simulink model "GuidanceLaw"  (R2023b)
settings: Solver=ode4  StartTime=0.0  StopTime=400  FixedStep=0.05  RelTol=1e-3
values from neighbouring files (symbols this model uses):
  APCMD_TYPE : value not decoded    [apDataDictionary.sldd]
  missionRoutePlan_struct = struct(      'validWpNum_u8', uint8(5),      'missionRoute_struct', repmat(wpDefault_struct, double(maxWpNum_u8), 1))    [initMissionRoutePlan_MC.m]
  MSSN_TYPE : value not decoded    [apDataDictionary.sldd]
  setPoint_struct = struct('lat_deg_d',double(31.200000),'lon_deg_d',double(121.500000),'alt_m_f',single(100),'yaw_deg_f',single(0))    [APTest.m]
undefined symbols (not defined in the file or in its folder): apParams
libraries: simulink x13, simulink_extras x3
(part 5 of 7)

== matlab function GuidanceLaw/Subsystem/wpMssnHandle/CrsTransform/geoToLocalNEU ==
  data: curGeo_struct input; curPosNEU_m_f output; preWpGeo_struct input; curWpGeo_struct input; nextWpGeo_struct input; segSwitch_b input; preWpNEU_m_f output; curWpNEU_m_f output; nextWpNEU_m_f output; newOriOldNEU_m_f output
function [curPosNEU_m_f, preWpNEU_m_f, curWpNEU_m_f, nextWpNEU_m_f, newOriOldNEU_m_f] = geoToLocalNEU(curGeo_struct, preWpGeo_struct, curWpGeo_struct, ...
    nextWpGeo_struct, segSwitch_b)
%#codegen
%
% 功能：
% 1. 以当前执行航点作为局部NEU坐标系原点；
% 2. 将当前位置、上一航点、当前航点和下一航点转换到局部NEU；
% 3. 航段切换时计算新原点在旧局部坐标系中的位置。
%
% 输入经纬高结构体字段：
% lat_deg_d：纬度，deg，double；
% lon_deg_d：经度，deg，double；
% alt_m_f：高度，m，single。

%% 保存上一周期实际使用的局部坐标原点

persistent lastOriginLat_deg_d
persistent lastOriginLon_deg_d
persistent lastOriginAlt_m_f
persistent originInitialized_b

if isempty(originInitialized_b)
    lastOriginLat_deg_d = double(0.0);
    lastOriginLon_deg_d = double(0.0);
    lastOriginAlt_m_f = single(0.0);
    originInitialized_b = false;
end


%% 当前局部坐标系原点

originLL_deg_d = [curWpGeo_struct.lat_deg_d, curWpGeo_struct.lon_deg_d];

originAlt_m_f = curWpGeo_struct.alt_m_f;

if ~originInitialized_b
    % 第一次运行没有旧坐标系，此时不需要平移轨迹状态
    lastOriginLat_deg_d = originLL_deg_d(1);
    lastOriginLon_deg_d = originLL_deg_d(2);
    lastOriginAlt_m_f = originAlt_m_f;
    originInitialized_b = true;
end

%% 飞机当前位置

curLL_deg_d = [curGeo_struct.lat_deg_d, curGeo_struct.lon_deg_d];

curPosNE_m_f = getDistanceNE(originLL_deg_d, curLL_deg_d);

curPosNEU_m_f = single(zeros(3,1));
curPosNEU_m_f(1) = curPosNE_m_f(1);
curPosNEU_m_f(2) = curPosNE_m_f(2);
curPosNEU_m_f(3) = curGeo_struct.alt_m_f - originAlt_m_f;

%% 上一航点

preWpLL_deg_d = [preWpGeo_struct.lat_deg_d, preWpGeo_struct.lon_deg_d];

preWpNE_m_f = getDistanceNE(originLL_deg_d, preWpLL_deg_d);

preWpNEU_m_f = single(zeros(3,1));
preWpNEU_m_f(1) = preWpNE_m_f(1);
preWpNEU_m_f(2) = preWpNE_m_f(2);
preWpNEU_m_f(3) = preWpGeo_struct.alt_m_f - originAlt_m_f;

%% 当前执行航点

% 当前执行航点就是局部坐标系原点。
curWpNEU_m_f = single(zeros(3,1));

%% 下一航点

nextWpLL_deg_d = [nextWpGeo_struct.lat_deg_d, nextWpGeo_struct.lon_deg_d];

nextWpNE_m_f = getDistanceNE(originLL_deg_d, nextWpLL_deg_d);

nextWpNEU_m_f = single(zeros(3,1));
nextWpNEU_m_f(1) = nextWpNE_m_f(1);
nextWpNEU_m_f(2) = nextWpNE_m_f(2);
nextWpNEU_m_f(3) = nextWpGeo_struct.alt_m_f - originAlt_m_f;

%% 新原点在旧局部坐标系中的位置

newOriOldNEU_m_f = single(zeros(3,1));

if segSwitch_b
    oldOriginLL_deg_d = [lastOriginLat_deg_d, lastOriginLon_deg_d];

    newOriginOldNE_m_f = getDistanceNE(oldOriginLL_deg_d, originLL_deg_d);

    newOriOldNEU_m_f(1) = single(newOriginOldNE_m_f(1));
    newOriOldNEU_m_f(2) = single(newOriginOldNE_m_f(2));
    newOriOldNEU_m_f(3) = originAlt_m_f - lastOriginAlt_m_f;
end

%% 保存本周期实际原点，供下一次切换使用

lastOriginLat_deg_d = originLL_deg_d(1);
lastOriginLon_deg_d = originLL_deg_d(2);
lastOriginAlt_m_f = originAlt_m_f;

end

== matlab function GuidanceLaw/Subsystem/wpMssnHandle/WpUpdate/WaypointSelector ==
  data: route_struct input; preWp_struct output Bus: wayPointBus; validWpNum_u8 input; curWpIdx_u8 input; curWp_struct output Bus: wayPointBus; nextWp_struct output Bus: wayPointBus
function [preWp_struct, curWp_struct, nextWp_struct] = WaypointSelector(route_struct, validWpNum_u8, curWpIdx_u8)
%#codegen
preWp_struct  = route_struct(1);
curWp_struct  = route_struct(1);
nextWp_struct = route_struct(1);

% 要求初始执行航点序列为2
if validWpNum_u8 < uint8(2) || curWpIdx_u8 < uint8(2)
    preWp_struct.wpType_u8  = WP_TYPE.INVALID_WP;
    curWp_struct.wpType_u8  = WP_TYPE.INVALID_WP;
    nextWp_struct.wpType_u8 = WP_TYPE.INVALID_WP;
    return;
end

idx_d = min(curWpIdx_u8,validWpNum_u8);
preWp_struct = route_struct(idx_d - uint8(1));
curWp_struct = route_struct(idx_d);

if idx_d < validWpNum_u8
    nextWp_struct = route_struct(idx_d + uint8(1));
else 
    nextWp_struct = curWp_struct;
    nextWp_struct.wpType_u8 = WP_TYPE.INVALID_WP;
end
end

== matlab function GuidanceLaw/Subsystem/wpMssnHandle/WaypointArrivalState/hoverPosJudge/conditionHoldJudge ==
  data: condition_b input; hoverPosJudge_b output; reset_b input; dt_s_f input; holdTimeCond_s_f input
function hoverPosJudge_b = conditionHoldJudge(condition_b, reset_b, dt_s_f, holdTimeCond_s_f)
%#codegen
%
% 条件连续保持时间判定
%
% 输入：
% condition_b           当前周期原始综合条件；
% reset_b               航段切换复位信号；
% dt_s_f                函数运行周期，s；
% holdTimeCond_s_f      条件需要连续保持的时间，s。
%
% 输出：
% hoverPosJudge_b       条件连续保持时间满足标志。

persistent holdElapsedTimeState_s_f

%% 状态初始化
if isempty(holdElapsedTimeState_s_f)
    holdElapsedTimeState_s_f = single(0.0);
end

%% 输入保护
dtValid_s_f = max(single(dt_s_f), single(0.0));
holdTimeValid_s_f = max(single(holdTimeCond_s_f), single(0.0));

%% 复位内部历史状态
if reset_b
    holdElapsedTimeState_s_f = single(0.0);
end

%% 本周期条件更新
if ~condition_b
    % 条件不成立，连续保持过程立即中断
    holdElapsedTimeState_s_f = single(0.0);
    hoverPosJudge_b = false;

elseif holdTimeValid_s_f <= single(0.0)
    % 无保持时间要求，当前周期条件成立即满足
    holdElapsedTimeState_s_f = single(0.0);
    hoverPosJudge_b = true;

else
    % 当前周期条件成立，立即累计一个执行周期
    elapsedTimeNext_s_f = holdElapsedTimeState_s_f + dtValid_s_f;

    % 达到目标时间后饱和，避免持续累加
    if elapsedTimeNext_s_f >= holdTimeValid_s_f
        holdElapsedTimeState_s_f = holdTimeValid_s_f;
        hoverPosJudge_b = true;
    else
        holdElapsedTimeState_s_f = elapsedTimeNext_s_f;
        hoverPosJudge_b = false;
    end
end

end

== stateflow chart GuidanceLaw/Subsystem/wpMssnHandle/WaypointArrivalState/ArrivalJudgeSelect ==
  state ACTIVE
    entry:
    judgeMethod_u8 = uint8(0);
    hoverPosJudgeEn_b = false;
    hoverYawJudgeEn_b = false;
    mcLineJudgeEn_b = false;
    fwLineJudgeEn_b = false;
    cirJudgeEn_b = false;
    state HOVER_POSITION
      entry:
      judgeMethod_u8 = uint8(1);
      hoverPosJudgeEn_b = true;
    note: 偏航角类型
        | 0：航向对准
        | 1：航点指定
        | 2：指向航点
    state HOVER_YAW_ALIGN
      entry:
      judgeMethod_u8 = uint8(2);
      hoverYawJudgeEn_b = true;
    state MC_LINE
      entry:
      judgeMethod_u8 = uint8(3);
      mcLineJudgeEn_b = true;
    state FW_LINE
      entry:
      judgeMethod_u8 = uint8(4);
      fwLineJudgeEn_b = true;
    state FW_CIR
      entry:
      judgeMethod_u8 = uint8(5);
      cirJudgeEn_b = true;
    state INVALID
      entry:
      judgeMethod_u8 = uint8(0);
    (junction 34) -> HOVER_POSITION [order 1] : [(curWp_struct.wpType_u8 == WP_TYPE.MC_TAKEOFF_WP && mssnType_u8 == MSSN_TYPE.VERTICAL_TAKEOFF) ||...
        |  (curWp_struct.wpType_u8 == WP_TYPE.MC_LAND_WP && preWp_struct.wpType_u8 ~= WP_TYPE.MC_LAND_WP)]
    (junction 34) -> HOVER_YAW_ALIGN [order 2] : [(curWp_struct.wpType_u8 == WP_TYPE.MC_TAKEOFF_WP && mssnType_u8 == MSSN_TYPE.ROUTE_FLIGHT) ||...
        | (curWp_struct.wpType_u8 == WP_TYPE.MC_LINE_WP && curWp_struct.fastWp_b == false)]
    (default) -> (junction 34)
    (junction 34) -> MC_LINE [order 3] : [curWp_struct.wpType_u8 == WP_TYPE.MC_LINE_WP && curWp_struct.fastWp_b == true]
    (junction 34) -> FW_LINE [order 4] : [curWp_struct.wpType_u8 == WP_TYPE.FW_LINE_WP &&...
        | mssnType_u8 ~=MSSN_TYPE.AUTO_FORWARD_TILT]
    (junction 34) -> FW_CIR [order 5] : [curWp_struct.wpType_u8 == WP_TYPE.FW_CIR_WP]
    (junction 34) -> INVALID [order 6]
  (default) -> ACTIVE
  ACTIVE -> ACTIVE : [segSwitch_b]
  data: curWp_struct input Bus: localNEUWpBus size=1; mssnType_u8 input size=1; segSwitch_b input boolean size=1; judgeMethod_u8 output uint8 size=1; hoverPosJudgeEn_b output boolean size=1; hoverYawJudgeEn_b output boolean size=1; mcLineJudgeEn_b output boolean size=1; fwLineJudgeEn_b output boolean size=1; cirJudgeEn_b output boolean size=1; nextWp_struct input Bus: localNEUWpBus size=1; preWp_struct input Bus: localNEUWpBus size=1

== matlab function GuidanceLaw/Subsystem/wpMssnHandle/WaypointArrivalState/hoverYawJudge/conditionHoldJudge ==
  data: condition_b input; hoverPosJudge_b output; reset_b input; dt_s_f input; holdTimeCond_s_f input
function hoverPosJudge_b = conditionHoldJudge(condition_b, reset_b, dt_s_f, holdTimeCond_s_f)
%#codegen
%
% 条件连续保持时间判定
%
% 输入：
% condition_b           当前周期原始综合条件；
% reset_b               航段切换复位信号；
% dt_s_f                函数运行周期，s；
% holdTimeCond_s_f      条件需要连续保持的时间，s。
%
% 输出：
% hoverPosJudge_b       条件连续保持时间满足标志。

persistent holdElapsedTimeState_s_f

%% 状态初始化
if isempty(holdElapsedTimeState_s_f)
    holdElapsedTimeState_s_f = single(0.0);
end

%% 输入保护
dtValid_s_f = max(single(dt_s_f), single(0.0));
holdTimeValid_s_f = max(single(holdTimeCond_s_f), single(0.0));

%% 复位内部历史状态
if reset_b
    holdElapsedTimeState_s_f = single(0.0);
end

%% 本周期条件更新
if ~condition_b
    % 条件不成立，连续保持过程立即中断
    holdElapsedTimeState_s_f = single(0.0);
    hoverPosJudge_b = false;

elseif holdTimeValid_s_f <= single(0.0)
    % 无保持时间要求，当前周期条件成立即满足
    holdElapsedTimeState_s_f = single(0.0);
    hoverPosJudge_b = true;

else
    % 当前周期条件成立，立即累计一个执行周期
    elapsedTimeNext_s_f = holdElapsedTimeState_s_f + dtValid_s_f;

    % 达到目标时间后饱和，避免持续累加
    if elapsedTimeNext_s_f >= holdTimeValid_s_f
        holdElapsedTimeState_s_f = holdTimeValid_s_f;
        hoverPosJudge_b = true;
    else
        holdElapsedTimeState_s_f = elapsedTimeNext_s_f;
        hoverPosJudge_b = false;
    end
end

end

== stateflow chart GuidanceLaw/Subsystem/wpMssnHandle/WaypointArrivalState/hoverYawJudge/HoverPosReachStateflow ==
  state WAIT_POSITION
    entry:
    isHoverPosReach_b = false;
  state POS_REACHED
    entry:
    isHoverPosReach_b = true;
  (default) -> (junction 13)
  (junction 13) -> POS_REACHED [order 1] : [hoverPosJudge_b]
  (junction 13) -> WAIT_POSITION [order 2]
  POS_REACHED -> (junction 13) : [reset_b]
  WAIT_POSITION -> POS_REACHED : [hoverPosJudge_b]
  data: hoverPosJudge_b input boolean size=1; reset_b input boolean size=1; isHoverPosReach_b output boolean size=1

== matlab function GuidanceLaw/Subsystem/wpMssnHandle/WaypointArrivalState/hoverYawJudge/YawAlignJudge/YawJudgeAlgorithmBlock ==
  data: curPosNE_m_f input; nextWpNE_m_f input; hoverYawJudge_b output boolean; curYaw_deg_f input; nextWpYawType_u8 input; nextWpYaw_deg_f input; reset_b input; dt_s_f input; yawErrAccept_deg_f input; holdTimeYaw_s_f input; minYawDirDist_m_f input; yawCmd_deg_f output; curWpNE_m_f input
function [hoverYawJudge_b, yawCmd_deg_f] = hoverYawAlignJudge(curPosNE_m_f, nextWpNE_m_f, curYaw_deg_f, nextWpYawType_u8, nextWpYaw_deg_f, reset_b, dt_s_f, ...
    yawErrAccept_deg_f, holdTimeYaw_s_f, minYawDirDist_m_f, curWpNE_m_f)
%#codegen
%
% 悬停位置到达后的目标航向生成与航向对准判定
%
% 下一航点偏航角类型：
% 0：航向对准——当前航点指向下一航点；
% 1：指向航点——位置到达时飞机位置指向下一航点；
% 2：航点指定——下一航点设定的偏航角。

persistent yawCmdState_deg_f
persistent yawCmdLockedState_b
persistent yawHoldTimeState_s_f
persistent yawReachedState_b

%% 状态初始化
if isempty(yawCmdState_deg_f)
    yawCmdState_deg_f = single(0.0);
    yawCmdLockedState_b = false;
    yawHoldTimeState_s_f = single(0.0);
    yawReachedState_b = false;
end

%% 参数保护
dtValid_s_f = max(dt_s_f, single(0.0));

yawErrAcceptValid_deg_f = min(max(yawErrAccept_deg_f, single(0.0)), single(180.0));

holdTimeYawValid_s_f = max(holdTimeYaw_s_f, single(0.0));

minYawDirDistValid_m_f = max(minYawDirDist_m_f, single(0.0));

%% 航段切换复位
% 只清除旧状态，随后仍处理当前拍。
if reset_b
    yawCmdState_deg_f = cldWrap180(curYaw_deg_f);
    yawCmdLockedState_b = false;
    yawHoldTimeState_s_f = single(0.0);
    yawReachedState_b = false;
end

%% 目标航向计算与锁存
if ~yawCmdLockedState_b

    % 位置首次到达，仅在当前拍计算一次目标航向。
    switch uint8(nextWpYawType_u8)

        case uint8(0)
            %% 航向对准
            % 当前航点为局部坐标系原点。
            yawDirN_m_f = nextWpNE_m_f(1) - curWpNE_m_f(1);
            yawDirE_m_f = nextWpNE_m_f(2) - curWpNE_m_f(2);

            yawCmdState_deg_f = directionNEToYaw(yawDirN_m_f, yawDirE_m_f, curYaw_deg_f, minYawDirDistValid_m_f);

        case uint8(1)
            %% 航点指定
            yawCmdState_deg_f = cldWrap180(nextWpYaw_deg_f);

        case uint8(2)

            %% 指向航点
            % 使用位置到达当前拍的飞机位置计算一次。
            yawDirN_m_f = nextWpNE_m_f(1) - curPosNE_m_f(1);

            yawDirE_m_f = nextWpNE_m_f(2) - curPosNE_m_f(2);

            yawCmdState_deg_f = directionNEToYaw(yawDirN_m_f, yawDirE_m_f, curYaw_deg_f, minYawDirDistValid_m_f);
            
        otherwise
            %% 无效偏航类型
            yawCmdState_deg_f = cldWrap180(curYaw_deg_f);
    end

    % 目标航向计算完成后立即锁存。
    yawCmdLockedState_b = true;
end

%% 输出锁存后的目标航向
yawCmd_deg_f = yawCmdState_deg_f;

%% 航向误差计算
yawErr_deg_f = cldWrap180(yawCmdState_deg_f - curYaw_deg_f);

yawCondition_b = yawCmdLockedState_b && abs(yawErr_deg_f) <= yawErrAcceptValid_deg_f;

%% 航向连续保持判定
if ~yawReachedState_b

    if ~yawCondition_b
        yawHoldTimeState_s_f = single(0.0);

    elseif holdTimeYawValid_s_f <= single(0.0)
        yawReachedState_b = true;

    else
        % 当前拍满足条件，立即累计一个dt。
        yawHoldTimeState_s_f = min(yawHoldTimeState_s_f + dtValid_s_f, holdTimeYawValid_s_f);

        yawReachedState_b = yawHoldTimeState_s_f >= holdTimeYawValid_s_f;
    end
end

%% 输出航向对准锁存结果
hoverYawJudge_b = yawReachedState_b;

end


function yaw_deg_f = directionNEToYaw(directionN_m_f, directionE_m_f, fallbackYaw_deg_f, minDirectionDist_m_f)
%#codegen
%
% NE方向向量转换为航向角：
% 北向0 deg，东向90 deg。

directionDistSq_m2_f = directionN_m_f * directionN_m_f + directionE_m_f * directionE_m_f;

minDirectionDistSq_m2_f = minDirectionDist_m_f * minDirectionDist_m_f;

if directionDistSq_m2_f > minDirectionDistSq_m2_f
    radToDeg_f = single(180.0 / pi);

    yaw_deg_f = atan2(directionE_m_f, directionN_m_f) * radToDeg_f;

    yaw_deg_f = cldWrap180(yaw_deg_f);
else
    % 水平向量过小，保持位置到达时的当前航向。
    yaw_deg_f = cldWrap180(single(fallbackYaw_deg_f));
end

end

== matlab function GuidanceLaw/Subsystem/wpMssnHandle/WaypointArrivalState/mcLineJudge/JudgeAlgorithm ==
  data: curPosNE_m_f input; mcLineJudge_b output; preWpNE_m_f input; curWpNE_m_f input; nextWpNE_m_f input; maxRouteSpeed_mps_f input; maxLatAcc_mps2_f input; minJudgeDist_m_f input; maxJudgeDist_m_f input; segmentLimitRatio_f input; reset_b input
function mcLineJudge_b = mcLineJudge(curPosNE_m_f, preWpNE_m_f, curWpNE_m_f, nextWpNE_m_f, maxRouteSpeed_mps_f, maxLatAcc_mps2_f, minJudgeDist_m_f, maxJudgeDist_m_f, segmentLimitRatio_f, reset_b)
%#codegen
%
% 旋翼直线航点提前分界面判定。
%
% 与轨迹生成器共用computeMcTurnConstraint：
% 1. maxRouteSpeed_mps_f只作为最大速度，不再作为固定转弯速度；
% 2. 根据A-B-C转角、横向加速度和可用提前距离计算动态航点通过速度；
% 3. 本模块仅使用其中的judgeDist_m_f确定分界面；
% 4. 轨迹生成器使用同一judgeDist和passSpeed提前减速，二者保持一致。
%
% geometryState_f：
% 1 提前判定距离，m
% 2 A->B单位方向北向分量
% 3 A->B单位方向东向分量
% 4 B点在A->B单位方向上的投影，m

persistent completeState_b
persistent geometryState_f
persistent initialized_b

smallValue_m_f = single(0.001);

if isempty(initialized_b)
    completeState_b = false;
    geometryState_f = single(zeros(4,1));
    initialized_b = false;
end

%% 新航段几何计算并冻结
if reset_b || ~initialized_b
    completeState_b = false;
    geometryState_f = single(zeros(4,1));

    inVecNE_m_f = curWpNE_m_f - preWpNE_m_f;
    inLength_m_f = norm(inVecNE_m_f);
    shortLineThreshold_m_f = max(max(minJudgeDist_m_f, single(0.0)), smallValue_m_f);

    if inLength_m_f <= shortLineThreshold_m_f
        % 当前航段太短，直接判定完成。
        completeState_b = true;
    else
        inDirNE_f = inVecNE_m_f / inLength_m_f;

        [judgeDist_m_f, ~] = computeMcTurnConstraint(preWpNE_m_f, curWpNE_m_f, nextWpNE_m_f, maxRouteSpeed_mps_f, maxLatAcc_mps2_f, ...
            minJudgeDist_m_f, maxJudgeDist_m_f, segmentLimitRatio_f, smallValue_m_f);

        geometryState_f(1) = judgeDist_m_f;
        geometryState_f(2) = inDirNE_f(1);
        geometryState_f(3) = inDirNE_f(2);
        geometryState_f(4) = dot(curWpNE_m_f, inDirNE_f);
    end

    initialized_b = true;
end

%% 使用冻结参数进行提前分界面判定
if ~completeState_b
    judgeDist_m_f = geometryState_f(1);
    inDirNE_f = geometryState_f(2:3);
    curWpAlong_m_f = geometryState_f(4);

    curPosAlong_m_f = dot(curPosNE_m_f, inDirNE_f);
    remainDist_m_f = curWpAlong_m_f - curPosAlong_m_f;

    if remainDist_m_f <= judgeDist_m_f
        completeState_b = true;
    end
end

% 完成后保持到下一次segSwitch/reset触发。
mcLineJudge_b = completeState_b;

end

== matlab function GuidanceLaw/Subsystem/wpMssnHandle/WaypointArrivalState/fwLineJudge/JudgeAlgorithm ==
  data: curPosNE_m_f input; fwLineJudge_b output; preWp_struct input; curWp_struct input; nextWp_struct input; turnRollPlan_deg_f input; effectRollRate_dps_f input; judgeDistMargin_f input; minJudgeDist_m_f input; maxJudgeDist_m_f input; segmentLimitRatio_f input; reset_b input; G_mps2_f input; cruiseAirSpd_mps_f input
function fwLineJudge_b = fwLineJudge(curPosNE_m_f, preWp_struct, curWp_struct, nextWp_struct, turnRollPlan_deg_f, effectRollRate_dps_f, ...
    judgeDistMargin_f, minJudgeDist_m_f, maxJudgeDist_m_f, segmentLimitRatio_f, reset_b, G_mps2_f, cruiseAirSpd_mps_f)
%#codegen
%
% 固定翼直线航点提前分界面判定
%
% 普通直线：
% Rplan = V^2 / (g * tan(turnRollPlan))
% Lraw  = Rplan * tan(turnAngle / 2)
% L     = judgeDistMargin * Lraw
%
% 圆弧：
% cirRoll  = atan(V^2 / (g * cirRadius))
% rollTime = cirRoll / effectRollRate
% L        = judgeDistMargin * V * rollTime
%
% geometryState_f：
% 1  冻结后的提前判定距离，m
% 2  A->B单位方向北向分量
% 3  A->B单位方向东向分量
% 4  B点在A->B单位方向上的投影，m

persistent completeState_b
persistent geometryState_f
persistent initState_b

smallValue_f = single(0.001);
zero_f = single(0.0);
one_f = single(1.0);
half_f = single(0.5);
degToRad_f = single(pi / 180.0);
maxAngle_rad_f = single(89.0) * degToRad_f;

preWpNE_m_f = [preWp_struct.posN_m_f; preWp_struct.posE_m_f];
curWpNE_m_f = [curWp_struct.posN_m_f; curWp_struct.posE_m_f];
nextWpNE_m_f = [nextWp_struct.posN_m_f; nextWp_struct.posE_m_f];

nextWpIsCir_b = nextWp_struct.wpType_u8 == WP_TYPE.FW_CIR_WP;

%% 持久状态初始化

if isempty(initState_b)
    completeState_b = false;
    geometryState_f = single(zeros(4, 1));
    initState_b = true;
end

%% 新航段几何参数计算与冻结

if initState_b || reset_b
    completeState_b = false;
    geometryState_f = single(zeros(4, 1));
    initState_b = false;

    % 当前航段A->B。
    inN_m_f = curWpNE_m_f(1) - preWpNE_m_f(1);
    inE_m_f = curWpNE_m_f(2) - preWpNE_m_f(2);

    % 下一航段B->C。
    outN_m_f = nextWpNE_m_f(1) - curWpNE_m_f(1);
    outE_m_f = nextWpNE_m_f(2) - curWpNE_m_f(2);

    inLength_m_f = sqrt(inN_m_f * inN_m_f + inE_m_f * inE_m_f);
    outLength_m_f = sqrt(outN_m_f * outN_m_f + outE_m_f * outE_m_f);

    minDist_m_f = max(minJudgeDist_m_f, zero_f);
    maxDist_m_f = max(maxJudgeDist_m_f, minDist_m_f);
    segmentRatio_f = min(max(segmentLimitRatio_f, zero_f), single(0.49));
    distanceMargin_f = max(judgeDistMargin_f, one_f);

    if inLength_m_f <= smallValue_f
        % 当前航段几何无效。
        completeState_b = true;

    else
        %% 当前航段方向

        inDirN_f = inN_m_f / inLength_m_f;
        inDirE_f = inE_m_f / inLength_m_f;

        %% 预计转弯速度

        if abs(curWp_struct.spd_mps_f) <= smallValue_f
            turnSpeed_mps_f = abs(cruiseAirSpd_mps_f);
        else
            turnSpeed_mps_f = abs(curWp_struct.spd_mps_f);
        end

        %% 转弯规划滚转角

        rollPlan_rad_f = abs(turnRollPlan_deg_f) * degToRad_f;
        rollPlan_rad_f = min(rollPlan_rad_f, maxAngle_rad_f);

        rawJudgeDist_m_f = minDist_m_f;

        if nextWpIsCir_b
            %% 下一航段为圆弧

            cirRadiusAbs_m_f = abs(nextWp_struct.radius_m_f);
            rollRateLimit_radps_f = abs(effectRollRate_dps_f) * degToRad_f;

            if cirRadiusAbs_m_f > smallValue_f

                % 当前转弯速度下跟踪圆弧所需的滚转角。
                cirRollDemand_rad_f = atan(turnSpeed_mps_f * turnSpeed_mps_f / (G_mps2_f * cirRadiusAbs_m_f));

                % 建立圆弧滚转角所需的时间。
                rollBuildTime_s_f = cirRollDemand_rad_f / rollRateLimit_radps_f;

                % 加入提前距离裕度。
                rawJudgeDist_m_f = distanceMargin_f * turnSpeed_mps_f * rollBuildTime_s_f;
            end

            % 下一航段为圆弧时，只使用当前直线长度限制。
            geometryMaxDist_m_f = segmentRatio_f * inLength_m_f;

        else
            %% 下一航段为普通直线

            if outLength_m_f > smallValue_f
                outDirN_f = outN_m_f / outLength_m_f;
                outDirE_f = outE_m_f / outLength_m_f;

                % 当前直线与下一直线之间的水平转角。
                turnDot_f = inDirN_f * outDirN_f + inDirE_f * outDirE_f;
                turnCross_f = inDirN_f * outDirE_f - inDirE_f * outDirN_f;

                turnDot_f = min(max(turnDot_f, -one_f), one_f);
                turnAngle_rad_f = atan2(abs(turnCross_f), turnDot_f);

                if rollPlan_rad_f > smallValue_f

                    % 规划使用的横向加速度。
                    planLatAcc_mps2_f = G_mps2_f * tan(rollPlan_rad_f);

                    if planLatAcc_mps2_f > smallValue_f
                        % 规划转弯半径，不再使用性能极限转弯半径。
                        planTurnRadius_m_f = turnSpeed_mps_f * turnSpeed_mps_f / planLatAcc_mps2_f;

                        halfTurnAngle_rad_f = half_f * turnAngle_rad_f;
                        halfTurnAngle_rad_f = min(halfTurnAngle_rad_f, maxAngle_rad_f);  % 夹角限制在89°

                        % 理论提前距离。
                        rawJudgeDist_m_f = planTurnRadius_m_f * tan(halfTurnAngle_rad_f);

                        % 对理论提前距离增加裕度。
                        rawJudgeDist_m_f = distanceMargin_f * rawJudgeDist_m_f;
                    end
                end

                % 同时受当前航段和下一航段长度限制。
                geometryMaxDist_m_f = segmentRatio_f * min(inLength_m_f, outLength_m_f);

            else
                % 下一航段几何无效。
                geometryMaxDist_m_f = segmentRatio_f * inLength_m_f;
            end
        end

        %% 提前距离统一限幅

        effectiveMaxDist_m_f = min(maxDist_m_f, geometryMaxDist_m_f);

        if effectiveMaxDist_m_f >= minDist_m_f
            judgeDist_m_f = min(max(rawJudgeDist_m_f, minDist_m_f), effectiveMaxDist_m_f);
        else
            judgeDist_m_f = effectiveMaxDist_m_f;
        end

        %% 冻结当前航段判定参数

        geometryState_f(1) = judgeDist_m_f;
        geometryState_f(2) = inDirN_f;
        geometryState_f(3) = inDirE_f;
        geometryState_f(4) = curWpNE_m_f(1) * inDirN_f + curWpNE_m_f(2) * inDirE_f;
    end
end

%% 提取冻结参数

judgeDist_m_f = geometryState_f(1);
inDirN_f = geometryState_f(2);
inDirE_f = geometryState_f(3);
curWpAlong_m_f = geometryState_f(4);

%% 提前分界面判定

if ~completeState_b
    curPosAlong_m_f = curPosNE_m_f(1) * inDirN_f + curPosNE_m_f(2) * inDirE_f;
    remainDist_m_f = curWpAlong_m_f - curPosAlong_m_f;

    if remainDist_m_f <= judgeDist_m_f
        completeState_b = true;
    end
end

%% 输出

fwLineJudge_b = completeState_b;

end

== matlab function GuidanceLaw/Subsystem/wpMssnHandle/WaypointArrivalState/cirJudge/MATLAB Function ==
  data: curPosNEU_m_f input; cirJudge_b output; curWpNEU_m_f input; nextWpNEU_m_f input; arrivalCond_u8 input; timeOrCount_u16 input; cirExitTolerance_deg_f input; cirAltTolerance_m_f input; dt_s_f input; reset_b input
function cirJudge_b = cirJudge(curPosNEU_m_f, curWpNEU_m_f, nextWpNEU_m_f, arrivalCond_u8, timeOrCount_u16, cirExitTolerance_deg_f, cirAltTolerance_m_f, dt_s_f, reset_b)
%#codegen
%
% 固定翼圆弧航点到达判定
%
% arrivalCond_u8：
% 0：方位角
% 1：时间 + 方位角，timeOrCount_u16单位为s
% 2：圈数 + 方位角，timeOrCount_u16单位为圈
% 3：高度 + 方位角
%
% 当前航点为圆心，下一航点确定圆弧切出方位角。
%
% 说明：
% orbitCountState_i32为-1表示尚未第一次进入切出扇区；
% 第一次进入切出扇区只作为圈数统计起点，不计为完成一圈。

persistent orbitTimeState_s_f
persistent orbitCountState_i32
persistent angleConditionPrevState_b

if isempty(orbitTimeState_s_f)
    orbitTimeState_s_f = single(0.0);
end

if isempty(orbitCountState_i32)
    orbitCountState_i32 = int32(-1);
end

if isempty(angleConditionPrevState_b)
    angleConditionPrevState_b = false;
end

%% 航段切换复位
% 只清除历史状态，不提前返回，当前拍继续参与判定

if reset_b
    orbitTimeState_s_f = single(0.0);
    orbitCountState_i32 = int32(-1);
    angleConditionPrevState_b = false;
end

%% 计算圆弧切出方位角条件

pN_m_f = curPosNEU_m_f(1) - curWpNEU_m_f(1);
pE_m_f = curPosNEU_m_f(2) - curWpNEU_m_f(2);

exitN_m_f = nextWpNEU_m_f(1) - curWpNEU_m_f(1);
exitE_m_f = nextWpNEU_m_f(2) - curWpNEU_m_f(2);

curBearing_rad_f = atan2(pE_m_f, pN_m_f);
exitBearing_rad_f = atan2(exitE_m_f, exitN_m_f);

angleErr_rad_f = atan2(sin(curBearing_rad_f - exitBearing_rad_f), cos(curBearing_rad_f - exitBearing_rad_f));
angleErr_deg_f = angleErr_rad_f * single(180.0 / pi);

angleTolerance_deg_f = max(single(cirExitTolerance_deg_f), single(0.0));
angleCondition_b = abs(angleErr_deg_f) <= angleTolerance_deg_f;

%% 计算高度条件

altitudeErr_m_f = curPosNEU_m_f(3) - curWpNEU_m_f(3);
altitudeTolerance_m_f = max(single(cirAltTolerance_m_f), single(0.0));
altitudeCondition_b = abs(altitudeErr_m_f) <= altitudeTolerance_m_f;

%% 附加条件判定

if arrivalCond_u8 == uint8(0)

    %% 方位角

    cirJudge_b = angleCondition_b;

elseif arrivalCond_u8 == uint8(1)

    %% 时间 + 方位角
    % reset_b当前拍清零后，仍累计当前拍的dt_s_f

    targetTime_s_f = single(timeOrCount_u16);
    validDt_s_f = max(single(dt_s_f), single(0.0));

    if orbitTimeState_s_f < targetTime_s_f
        orbitTimeState_s_f = orbitTimeState_s_f + validDt_s_f;
        orbitTimeState_s_f = min(orbitTimeState_s_f, targetTime_s_f);
    end

    cirJudge_b = orbitTimeState_s_f >= targetTime_s_f && angleCondition_b;

elseif arrivalCond_u8 == uint8(2)

    %% 圈数 + 方位角
    %
    % angleCondition_b的false->true表示飞机从切出扇区外
    % 重新进入切出扇区。
    %
    % 第一次进入：
    % orbitCountState_i32由-1变为0，只建立计圈起点。
    %
    % 后续每次重新进入：
    % orbitCountState_i32加1，表示完成一整圈。

    requiredOrbitCount_i32 = int32(max(timeOrCount_u16, uint16(1)));

    if angleCondition_b && ~angleConditionPrevState_b

        if orbitCountState_i32 < int32(0)
            orbitCountState_i32 = int32(0);
        else
            orbitCountState_i32 = orbitCountState_i32 + int32(1);
        end
    end

    angleConditionPrevState_b = angleCondition_b;

    cirJudge_b = orbitCountState_i32 >= requiredOrbitCount_i32 && angleCondition_b;

elseif arrivalCond_u8 == uint8(3)

    %% 高度 + 方位角

    cirJudge_b = altitudeCondition_b && angleCondition_b;
else
    %% 其它情况就按方位角来判断

    cirJudge_b = angleCondition_b;

end

end
